simulink model "setpoint_weighting_simulink"  (R2022a)
settings: Solver=VariableStepAuto  StartTime=0.0  StopTime=3500  RelTol=1e-3
undefined symbols (not defined in the file): K_sys, Kp, sigbuilder_block, tau_sys, Td, theta_sys, Ti
settings Model: Creator=raha  LastModifiedBy=raha

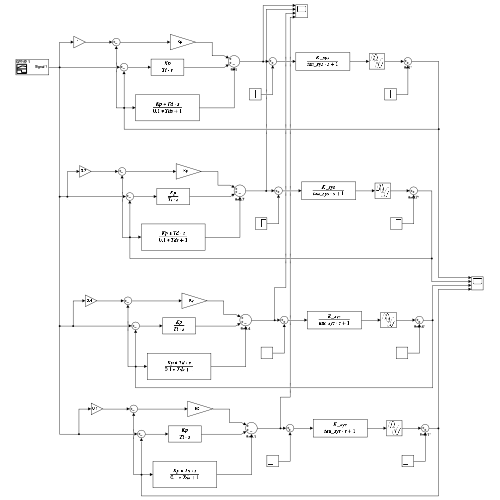
[thumbnail: Simulink's stored preview of the top-level diagram]
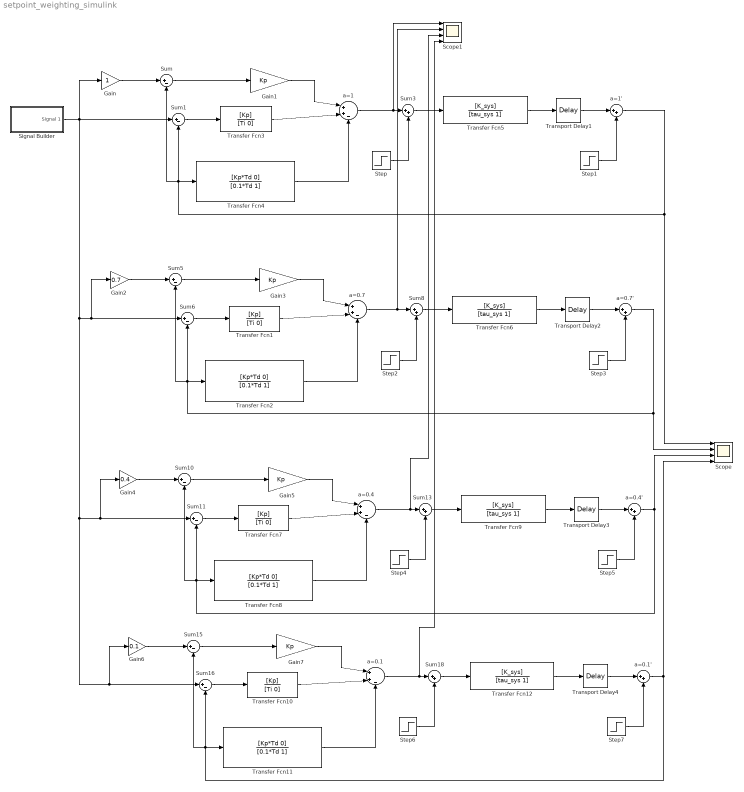
== system setpoint_weighting_simulink ==
  Gain : Gain
  Gain{1,3,5,7} (4 alike) : Gain  Gain=Kp
  Gain2 : Gain  Gain=0.7
  Gain4 : Gain  Gain=0.4
  Gain6 : Gain  Gain=0.1
  Scope : Scope  NumInputPorts=4
  Scope1 : Scope  NumInputPorts=4
  Signal Builder : Subsystem  Tag=STV Subsys  LoadFcn=sigbuilder_block('load');  StartFcn=sigbuilder_block('start');  StopFcn=sigbuilder_block('stop');  ClipboardFcn=sigbuilder_block('clipboard');  mask(Sigbuilder block){tuvar=[0:10]}
      mask help: Simulink:masks:SigbuilderBlock_MD
      mask init:
      | if ~strcmp(get_param(bdroot(gcbh),'SimulationStatus'),'stopped') tuvar = sigbuilder_block('maskInit'); end
      settings: CopyFcn=sigbuilder_block('copy');  DeleteFcn=sigbuilder_block('delete');  ModelCloseFcn=sigbuilder_block('modelClose');  PreSaveFcn=sigbuilder_block('preSave');  PauseFcn=sigbuilder_block('pause');  ContinueFcn=sigbuilder_block('continue');  NameChangeFcn=sigbuilder_block('namechange');  OpenFcn=sigbuilder_block('open',[437.6 199.2 550.4 400 ]);  CloseFcn=sigbuilder_block('close');
      mask Display: plot(0, 0, 100, 100,[2, 2, 32, 32, 2], [68, 8, 8, 68, 68],[32, 2], [38, 38], [32, 19, 2],[53, 60, 44], [32, 17, 17, 2],[16, 16, 31, 31]);txt = getActiveGroup(gcbh);text(2, 100, txt,'verticalAlignment', 'top');
  Step{,2,4,6} (4 alike) : Step  Time=1500  After=10  SampleTime=0
  Step{1,3,5,7} (4 alike) : Step  Time=2500  After=10  SampleTime=0
  Sum{,1,5..6,10..11,15..16} (8 alike) : Sum  Inputs=|+-
  Sum{3,8,13,18} (4 alike) : Sum  Inputs=|++
  Transfer Fcn{1,3,7,10} (4 alike) : TransferFcn  Numerator=[Kp]  Denominator=[Ti 0]
  Transfer Fcn{2,4,8,11} (4 alike) : TransferFcn  Numerator=[Kp*Td 0]  Denominator=[0.1*Td 1]
  Transfer Fcn{5..6,9,12} (4 alike) : TransferFcn  Numerator=[K_sys]  Denominator=[tau_sys 1]
  Transport Delay{1..4} (4 alike) : TransportDelay  DelayTime=theta_sys
  a=0.1 : Sum  Inputs=|++-
  a=0.1' : Sum  Inputs=|++
  a=0.4 : Sum  Inputs=|++-
  a=0.4' : Sum  Inputs=|++
  a=0.7 : Sum  Inputs=|++-
  a=0.7' : Sum  Inputs=|++
  a=1 : Sum  Inputs=|++-
  a=1' : Sum  Inputs=|++
  wires:
  Gain/1 -> Sum/1
  Sum/1 -> Gain1/1
  Sum1/1 -> Transfer Fcn3/1
  Transfer Fcn3/1 -> a=1/2
  Gain1/1 -> a=1/1
  Transfer Fcn4/1 -> a=1/3
  a=1/1 -> Scope1/1, Sum3/1
  Sum3/1 -> Transfer Fcn5/1
  Transfer Fcn5/1 -> Transport Delay1/1
  Transport Delay1/1 -> a=1'/1
  a=1'/1 -> Sum/2, Transfer Fcn4/1, Sum1/2, Scope/1
  Step/1 -> Sum3/2
  Step1/1 -> a=1'/2
  Sum5/1 -> Gain3/1
  Sum6/1 -> Transfer Fcn1/1
  Step2/1 -> Sum8/2
  Gain2/1 -> Sum5/1
  Transfer Fcn1/1 -> a=0.7/2
  Sum8/1 -> Transfer Fcn6/1
  Gain3/1 -> a=0.7/1
  a=0.7'/1 -> Sum5/2, Transfer Fcn2/1, Sum6/2, Scope/2
  Transfer Fcn6/1 -> Transport Delay2/1
  a=0.7/1 -> Sum8/1, Scope1/2
  Signal Builder/1(Signal 1) -> Gain4/1, Sum11/1, Gain6/1, Sum16/1, Gain2/1, Sum6/1, Sum1/1, Gain/1
  Step3/1 -> a=0.7'/2
  Transfer Fcn2/1 -> a=0.7/3
  Transport Delay2/1 -> a=0.7'/1
  Sum10/1 -> Gain5/1
  Step5/1 -> a=0.4'/2
  Sum13/1 -> Transfer Fcn9/1
  Step4/1 -> Sum13/2
  Gain5/1 -> a=0.4/1
  Transfer Fcn9/1 -> Transport Delay3/1
  Transport Delay3/1 -> a=0.4'/1
  a=0.4/1 -> Scope1/3, Sum13/1
  Transfer Fcn7/1 -> a=0.4/2
  Sum11/1 -> Transfer Fcn7/1
  Gain4/1 -> Sum10/1
  Transfer Fcn8/1 -> a=0.4/3
  a=0.4'/1 -> Sum10/2, Transfer Fcn8/1, Sum11/2, Scope/3
  Sum15/1 -> Gain7/1
  Step7/1 -> a=0.1'/2
  Sum18/1 -> Transfer Fcn12/1
  Step6/1 -> Sum18/2
  Gain7/1 -> a=0.1/1
  Transfer Fcn12/1 -> Transport Delay4/1
  Transport Delay4/1 -> a=0.1'/1
  a=0.1/1 -> Scope1/4, Sum18/1
  Transfer Fcn10/1 -> a=0.1/2
  Sum16/1 -> Transfer Fcn10/1
  Gain6/1 -> Sum15/1
  Transfer Fcn11/1 -> a=0.1/3
  a=0.1'/1 -> Sum15/2, Transfer Fcn11/1, Sum16/2, Scope/4

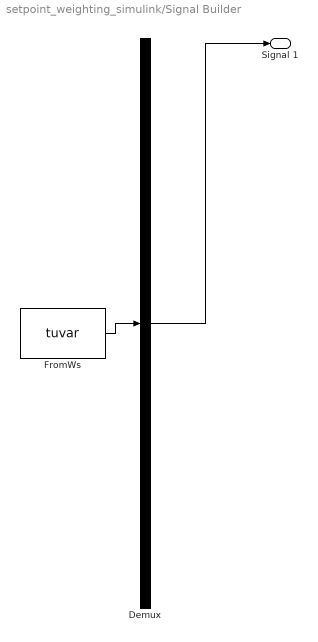
== system setpoint_weighting_simulink/Signal Builder ==
  Demux : Demux  Tag=STV Demux  Outputs=1
      settings: DisplayOption=none
  FromWs : FromWorkspace  Tag=STV FromWs  VariableName=tuvar
      SigBuilderData=|
      | common.afterFinalStr = 'Extrapolate'
      | common.sampleTime = 0
      | dataSet.timeRange = [0 3500]
      | dataSet.name = 'Group 1'
      | sbobj.Groups.Name = 'Group 1'
      | sbobj.Groups.Signals.Name = 'Signal 1'
      | sbobj.Groups.Signals.XData = [0 620 620 1630 1630 3500]
      | sbobj.Groups.Signals.YData = [35 35 55.2 55.2 45 45]
      | sbobj.Groups.TimeRange = [0 3500]
  Signal 1 : Outport  Tag=STV Outport
  wires:
  Demux/1 -> Signal 1/1
  FromWs/1 -> Demux/1
